simulink model "digital_communication_system_bpsk_80bit_backup"  (R2026b)
settings: Solver=VariableStepAuto  StopTime=1
undefined symbols (not defined in the file or in its folder): dcsim_txBits
settings Model: Creator=omarm  LastModifiedBy=omarm

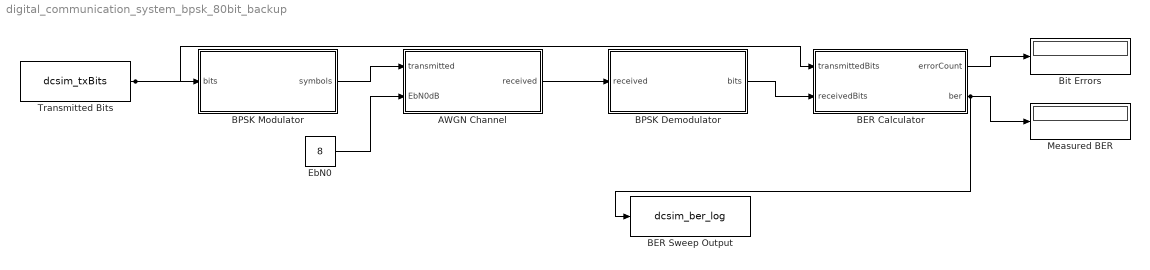
== system digital_communication_system_bpsk_80bit_backup ==
  AWGN Channel : MATLAB Function  TreatAsAtomicUnit=on
  BER Calculator : MATLAB Function  TreatAsAtomicUnit=on
  BER Sweep Output : ToWorkspace  VariableName=dcsim_ber_log  SampleTime=-1
  BPSK Demodulator : MATLAB Function  TreatAsAtomicUnit=on
  BPSK Modulator : MATLAB Function  TreatAsAtomicUnit=on
  Bit Errors : Display
  EbN0 : Constant  Value=8
  Measured BER : Display
  Transmitted Bits : Constant  Value=dcsim_txBits
  wires:
  Transmitted Bits/1 -> BPSK Modulator/1(bits), BER Calculator/1(transmittedBits)
  BPSK Modulator/1(symbols) -> AWGN Channel/1(transmitted)
  AWGN Channel/1(received) -> BPSK Demodulator/1(received)
  BPSK Demodulator/1(bits) -> BER Calculator/2(receivedBits)
  BER Calculator/1(errorCount) -> Bit Errors/1
  BER Calculator/2(ber) -> Measured BER/1, BER Sweep Output/1
  EbN0/1 -> AWGN Channel/2(EbN0dB)

== matlab function digital_communication_system_bpsk_80bit_backup/BPSK Modulator ==
  data: bits input; symbols output
function symbols = fcn(bits)
% Map binary 0 to +1 and binary 1 to -1.
symbols = 1 - 2*double(bits);
end

== matlab function digital_communication_system_bpsk_80bit_backup/BPSK Demodulator ==
  data: received input; bits output
function bits = fcn(received)
% Decide 0 for nonnegative samples and 1 for negative samples.
bits = double(received < 0);
end

== matlab function digital_communication_system_bpsk_80bit_backup/BER Calculator ==
  data: transmittedBits input; errorCount output; receivedBits input; ber output
function [errorCount, ber] = fcn(transmittedBits, receivedBits)
% Compare transmitted and received bits.
errors = transmittedBits ~= receivedBits;
errorCount = sum(errors);
ber = errorCount / numel(transmittedBits);
end

== matlab function digital_communication_system_bpsk_80bit_backup/AWGN Channel ==
  data: transmitted input; received output; EbN0dB input
function received = fcn(transmitted, EbN0dB)

EbN0 = 10^(EbN0dB/10);
noiseStd = sqrt(1/(2*EbN0));

received = transmitted + noiseStd*randn(size(transmitted));

end
